simulink model "quarter_car_model"  (R2026b)
settings: Solver=ode45  StopTime=45  MaxStep=0.001
PreLoadFcn:
  | road_ts = qc_road_input();
settings Model: Creator=rithvin007  LastModifiedBy=rithvin007

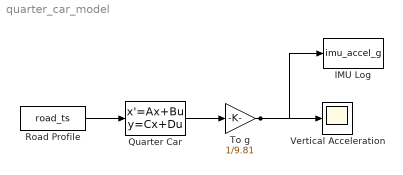
== system quarter_car_model ==
  IMU Log : ToWorkspace  VariableName=imu_accel_g  SaveFormat=Timeseries  SampleTime=-1
  Quarter Car : StateSpace  A=[0 1 0 0;-88.8888888888889 -4.44444444444444 88.8888888888889 4.44444444444444;0 0 0 1;800 40 -4400 -40]  B=[0;0;0;3600]  C=[-88.8888888888889 -4.44444444444444 88.8888888888889 4.44444444444444;800 40 -4400 -40]  D=[0;3600]  InitialCondition=[0;0;0;0]
  Road Profile : FromWorkspace  VariableName=road_ts  OutputAfterFinalValue=Holding final value
  To g : Gain  Gain=1/9.81
  Vertical Acceleration : Scope
  wires:
  To g/1 -> Vertical Acceleration/1, IMU Log/1
  Quarter Car/1 -> To g/1
  Road Profile/1 -> Quarter Car/1
